simulink model "DWPT_DD_4section_100V"  (R2026b)
settings: Solver=ode3  StopTime=.050  FixedStep=Ts
model workspace (MAT data in the model file):
  Cf = 1e-07
  Cout = 0.0022
  Cp = 2.26347657939e-08
  Cs = 1.84570546919e-08
  ESRf = 0.003
  ESRp = 0.005
  ESRs = 0.005
  Goff = 1e-08
  Ki = 15
  Kp = 0.012
  Lf = 4.05284734569e-06
  Lmat = [2.19582561429e-05  -4.36667057516e-08  -2.64487562385e-10  -2.91825501354e-11  1.6585415982e-06; -4.36667057516e-08  2.19582561429e-05  -4.36667057516e-08  -2.64487562385e-10  1.6585415982e-06; -2.64487562385e-10  -4.36667057516e-08  2.19582561429e-05  -4.36667057516e-08  -1.36008982282e-09; -2.91825501354e-11  -2.64487562385e-10  -4.36667057516e-08  2.19582561429e-05  -7.55518058561e-11; 1.6585415982e-06  1.6585415982e-06  -1.36008982282e-09  -7.55518058561e-11  2.19582561429e-05]
  QossTx = 1.45e-07
  RL = 3
  Rcoil = 0.019579897138
  Rf = 0.006
  RonSR = 0.0032
  RonTx = 0.008
  Ts = 1e-08
  Vdc = 100
  Vtarget = 60
  bodyRon = 0.01
  bodyRonTx = 0.008
  bodyVf = 0.8
  bodyVfTx = 2
  deadTime = 2e-08
  f = 250000
  initialOutputVoltage = 0
  position = 0.9144
  softStart = 0.02
  srDeadTime = 4e-08
  srEnabled = 1
  srThreshold = 0.25
  transitionTime = 5e-09
  u_nom = [0.744962860955 0.744962860955 0 0]
libraries: fl_lib x52, nesl_utility x42, ee_lib x20, ddtrack_lib x1
(part 1 of 4)
settings Model: Creator=rithvik  LastModifiedBy=rithvik
settings DataIOCC: SignalLogging=off
settings SimscapeCC: SimscapeLogType=all  SimscapeNominalValues="[{\"value\":\"1\",\"unit\":\"A\"},{\"value\":\"1\",\"unit\":\"bar\"},{\"value\":\"1\",\"unit\":\"cm^2\"},{\"value\":\"1\",\"unit\":\"cm^3/s\"},{\"value\":\"1\",\"unit\":\"kJ/kg\"},{\"value\":\"1\",\"unit\":\"kW\"},{\"value\":\"1\",\"unit\":\"l\"},{\"value\":\"1\",\"unit\":\"N\"},{\"value\":\"1\",\"unit\":\"N*m\"},{\"value\":\"1\",\"unit\":\"V\"},{\"value\":\"0.001\",\"unit\":\"Wb\"}]"  SimscapeUseEnergyAccounting=off

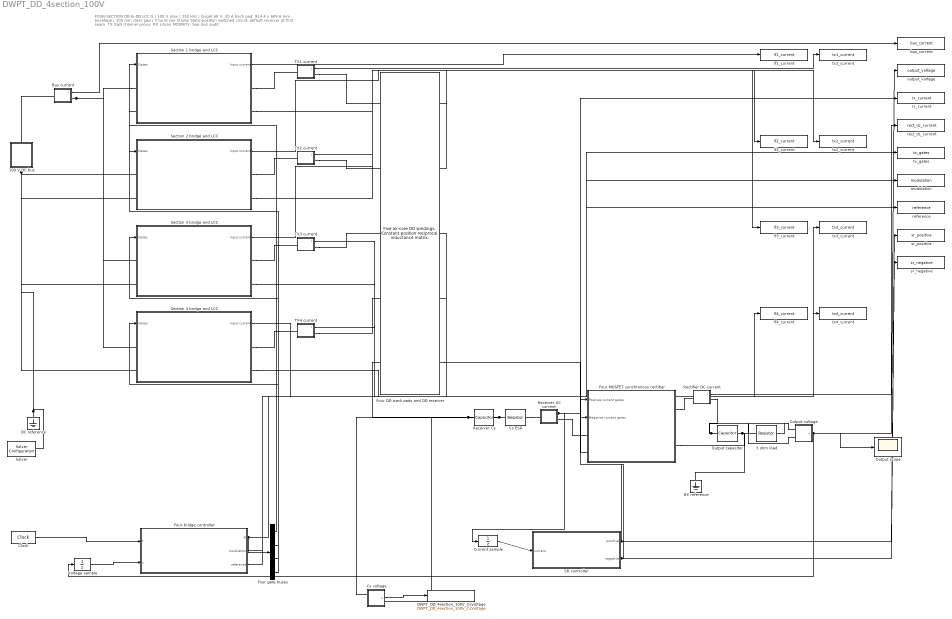
== system DWPT_DD_4section_100V ==
  note: FOUR-SECTION DD-to-DD LCC-S | 100 V max | 250 kHz | target 60 V, 20 A
      | Each pad: 914.4 x 609.6 mm envelope | 100 mm clear gap | 3 turns per D lobe
      | Static-position switched circuit; default receiver at first seam. TX GaN channel proxy; RX silicon MOSFETs. See loss audit.
  100 V DC bus : Subsystem
      settings: OpenFcn=elec.conv.unmask(gcb);
  3 ohm load : fl_lib/Electrical/Electrical Elements/Resistor  R=RL Ohm  i_specify=off  i_priority=None  i=0 A  i_nominal_specify=off  i_nominal_value=1  i_nominal_unit=A  v_specify=off  v_priority=None  v=0 V  v_nominal_specify=off  v_nominal_value=1  v_nominal_unit=V
  Bus current : Subsystem
      settings: OpenFcn=elec.conv.unmask(gcb);
  Clock : DigitalClock  SampleTime=Ts
  Cs ESR : fl_lib/Electrical/Electrical Elements/Resistor  R=ESRs Ohm  i_specify=off  i_priority=None  i=0 A  i_nominal_specify=off  i_nominal_value=1  i_nominal_unit=A  v_specify=off  v_priority=None  v=0 V  v_nominal_specify=off  v_nominal_value=1  v_nominal_unit=V
  Cs voltage : Subsystem
      settings: OpenFcn=elec.conv.unmask(gcb);
  Current sample : UnitDelay  SampleTime=Ts
  DC reference : fl_lib/Electrical/Electrical Elements/Electrical Reference
  DWPT_DD_4section_100V_CsVoltage : ToWorkspace  VariableName=DWPT_DD_4section_100V_CsVoltage  SaveFormat=Timeseries  SampleTime=-1
      settings: Decimation=max(1,round(20e-9/Ts))
  Four DD track pads and DD receiver : ddtrack_lib/Five air-core DD windings. Constant-position reciprocal inductance matrix.  Lmat=Lmat H  Rw=Rcoil Ohm  i1_specify=off  i1_priority=High  i1=0 A  i1_nominal_specify=off  i1_nominal_value=1  i1_nominal_unit=A  i2_specify=off  i2_priority=High  i2=0 A  i2_nominal_specify=off  i2_nominal_value=1  i2_nominal_unit=A  i3_specify=off  i3_priority=High  i3=0 A  i3_nominal_specify=off  i3_nominal_value=1  i3_nominal_unit=A  i4_specify=off  i4_priority=High  i4=0 A  i4_nominal_specify=off  i4_nominal_value=1  i4_nominal_unit=A  i5_specify=off  i5_priority=High  i5=0 A  i5_nominal_specify=off  i5_nominal_value=1  i5_nominal_unit=A
  Four MOSFET synchronous rectifier : Subsystem
  Four bridge controller : MATLAB Function  TreatAsAtomicUnit=on
  Four gate buses : Demux  Outputs=[4 4 4 4]
  Output capacitor : fl_lib/Electrical/Electrical Elements/Capacitor  c=Cout F  r=1e-6 Ohm  g=0 1/Ohm  i_specify=off  i_priority=None  i=0 A  i_nominal_specify=off  i_nominal_value=1  i_nominal_unit=A  v_specify=off  v_priority=None  v=0 V  v_nominal_specify=off  v_nominal_value=1  v_nominal_unit=V  vc_specify=on  vc_priority=High  vc=initialOutputVoltage V  vc_nominal_specify=off  vc_nominal_value=1  vc_nominal_unit=V
  Output scope : Scope
  Output voltage : Subsystem
      settings: OpenFcn=elec.conv.unmask(gcb);
  RX reference : fl_lib/Electrical/Electrical Elements/Electrical Reference
  Receiver AC current : Subsystem
      settings: OpenFcn=elec.conv.unmask(gcb);
  Receiver Cs : fl_lib/Electrical/Electrical Elements/Capacitor  c=Cs F  r=1e-6 Ohm  g=0 1/Ohm  i_specify=off  i_priority=None  i=0 A  i_nominal_specify=off  i_nominal_value=1  i_nominal_unit=A  v_specify=off  v_priority=None  v=0 V  v_nominal_specify=off  v_nominal_value=1  v_nominal_unit=V  vc_specify=on  vc_priority=High  vc=0 V  vc_nominal_specify=off  vc_nominal_value=1  vc_nominal_unit=V
  Rectifier DC current : Subsystem
      settings: OpenFcn=elec.conv.unmask(gcb);
  SR controller : MATLAB Function  TreatAsAtomicUnit=on
  Section 1 bridge and LCC : Subsystem
  Section 2 bridge and LCC : Subsystem
  Section 3 bridge and LCC : Subsystem
  Section 4 bridge and LCC : Subsystem
  Solver : nesl_utility/Solver Configuration  PhysicalDomain=network_engine_domain  SubClassName=solver  LeftPortType=input  RightPortType=generic  Tones=[]  Harmonics=[]  SimulateNoise=off  Profile=off  UseLocalSampling=off  EnableSwitchedLinearOptims=on  FrequencyDomain=off  UseCCode=off  RelTol=0.001  AbsTol=0.001  MinStep=1e-09  ToWorkspace=off  RevertToSquareIcSolve=off  NumHomotopyIterations=100  PhasorMode=off  PhasorModeNumHarmonics=1  ConsistencySolver=NEWTON_XTOL_AFTER_FTOL  CanonicalOrdering=CANONICAL  OptimizeIntermediates=OPTIMIZED  MulticoreSolverChoice=BACKWARD_EULER  IndexReductionMethod=DerivativeReplacement  DoDC=off  ResidualTolerance=1e-09  ConsistencyTolSource=GLOBAL  ConsistencyAbsTol=0.001  ConsistencyRelTol=0.001  ConsistencyTolFactor=0.001  UseLocalSolver=on  LocalSolverChoice=NE_TRAPEZOIDAL_ADVANCER  ResolveIndetEquations=on  FunctionEvalNumThread=1  LocalSolverSampleTime=Ts  DoFixedCost=off  MaxNonlinIter=3  MaxModeIter=2  ComputeImpulses=off  ImpulseIterations=2  LinearAlgebra=auto  LinearAlgebraNumThread=0  EquationFormulation=NE_TIME_EF  DelaysMemoryBudget=1024  AutomaticFiltering=on  FilteringTimeConstant=0.001  PartitionStorageMethod=AS_NEEDED  PartitionMemoryBudget=1024  PartitionMethod=BALANCED  MultibodyUseLocalSolver=off  MultibodyLocalSolverChoice=ODE1  MultibodyLocalSolverSampleTime=0.001
  TX1 current : Subsystem
      settings: OpenFcn=elec.conv.unmask(gcb);
  TX2 current : Subsystem
      settings: OpenFcn=elec.conv.unmask(gcb);
  TX3 current : Subsystem
      settings: OpenFcn=elec.conv.unmask(gcb);
  TX4 current : Subsystem
      settings: OpenFcn=elec.conv.unmask(gcb);
  Voltage sample : UnitDelay  SampleTime=Ts
  bus_current : ToWorkspace  VariableName=bus_current  SaveFormat=Timeseries  SampleTime=-1
  lf1_current : ToWorkspace  VariableName=lf1_current  SaveFormat=Timeseries  SampleTime=-1
      settings: Decimation=max(1,round(20e-9/Ts))
  lf2_current : ToWorkspace  VariableName=lf2_current  SaveFormat=Timeseries  SampleTime=-1
      settings: Decimation=max(1,round(20e-9/Ts))
  lf3_current : ToWorkspace  VariableName=lf3_current  SaveFormat=Timeseries  SampleTime=-1
      settings: Decimation=max(1,round(20e-9/Ts))
  lf4_current : ToWorkspace  VariableName=lf4_current  SaveFormat=Timeseries  SampleTime=-1
      settings: Decimation=max(1,round(20e-9/Ts))
  modulation : ToWorkspace  VariableName=modulation  SaveFormat=Timeseries  SampleTime=-1
      settings: Decimation=max(1,round(20e-9/Ts))
  output_voltage : ToWorkspace  VariableName=output_voltage  SaveFormat=Timeseries  SampleTime=-1
      settings: Decimation=max(1,round(20e-9/Ts))
  rect_dc_current : ToWorkspace  VariableName=rect_dc_current  SaveFormat=Timeseries  SampleTime=-1
      settings: Decimation=max(1,round(20e-9/Ts))
  reference : ToWorkspace  VariableName=reference  SaveFormat=Timeseries  SampleTime=-1
      settings: Decimation=max(1,round(20e-9/Ts))
  rx_current : ToWorkspace  VariableName=rx_current  SaveFormat=Timeseries  SampleTime=-1
      settings: Decimation=max(1,round(20e-9/Ts))
  sr_negative : ToWorkspace  VariableName=sr_negative  SaveFormat=Timeseries  SampleTime=-1
      settings: Decimation=max(1,round(20e-9/Ts))
  sr_positive : ToWorkspace  VariableName=sr_positive  SaveFormat=Timeseries  SampleTime=-1
      settings: Decimation=max(1,round(20e-9/Ts))
  tx1_current : ToWorkspace  VariableName=tx1_current  SaveFormat=Timeseries  SampleTime=-1
      settings: Decimation=max(1,round(20e-9/Ts))
  tx2_current : ToWorkspace  VariableName=tx2_current  SaveFormat=Timeseries  SampleTime=-1
      settings: Decimation=max(1,round(20e-9/Ts))
  tx3_current : ToWorkspace  VariableName=tx3_current  SaveFormat=Timeseries  SampleTime=-1
      settings: Decimation=max(1,round(20e-9/Ts))
  tx4_current : ToWorkspace  VariableName=tx4_current  SaveFormat=Timeseries  SampleTime=-1
      settings: Decimation=max(1,round(20e-9/Ts))
  tx_gates : ToWorkspace  VariableName=tx_gates  SaveFormat=Timeseries  SampleTime=-1
      settings: Decimation=max(1,round(20e-9/Ts))
  wires:
  Section 1 bridge and LCC/1(Input current) -> lf1_current/1
  TX1 current/1(i) -> tx1_current/1
  Section 2 bridge and LCC/1(Input current) -> lf2_current/1
  TX2 current/1(i) -> tx2_current/1
  Section 3 bridge and LCC/1(Input current) -> lf3_current/1
  TX3 current/1(i) -> tx3_current/1
  Section 4 bridge and LCC/1(Input current) -> lf4_current/1
  TX4 current/1(i) -> tx4_current/1
  Clock/1 -> Four bridge controller/1(t)
  Output voltage/1(v) -> Voltage sample/1, output_voltage/1, Output scope/1
  Voltage sample/1 -> Four bridge controller/2(v)
  Four bridge controller/1(g) -> Four gate buses/1, tx_gates/1
  Four gate buses/1 -> Section 1 bridge and LCC/1(Gates)
  Four gate buses/2 -> Section 2 bridge and LCC/1(Gates)
  Four gate buses/3 -> Section 3 bridge and LCC/1(Gates)
  Four gate buses/4 -> Section 4 bridge and LCC/1(Gates)
  Receiver AC current/1(i) -> Current sample/1, rx_current/1
  Current sample/1 -> SR controller/1(current)
  SR controller/1(positive) -> Four MOSFET synchronous rectifier/1(Positive current gates), sr_positive/1
  SR controller/2(negative) -> Four MOSFET synchronous rectifier/2(Negative current gates), sr_negative/1
  Bus current/1(i) -> bus_current/1
  Rectifier DC current/1(i) -> rect_dc_current/1
  Four bridge controller/2(modulation) -> modulation/1
  Four bridge controller/3(reference) -> reference/1
  Cs voltage/1(v) -> DWPT_DD_4section_100V_CsVoltage/1
  connections:
  100 V DC bus/RConn1 -- Bus current/LConn1
  DC reference/LConn1 -- 100 V DC bus/LConn1 -- Section 1 bridge and LCC/LConn2 -- Section 2 bridge and LCC/LConn2 -- Section 3 bridge and LCC/LConn2 -- Section 4 bridge and LCC/LConn2 -- Solver/RConn1
  Section 1 bridge and LCC/LConn1 -- Bus current/RConn1 -- Section 2 bridge and LCC/LConn1 -- Section 3 bridge and LCC/LConn1 -- Section 4 bridge and LCC/LConn1
  Section 1 bridge and LCC/RConn1 -- TX1 current/LConn1
  TX1 current/RConn1 -- Four DD track pads and DD receiver/LConn1
  Section 1 bridge and LCC/RConn2 -- Four DD track pads and DD receiver/RConn1
  Section 2 bridge and LCC/RConn1 -- TX2 current/LConn1
  TX2 current/RConn1 -- Four DD track pads and DD receiver/LConn2
  Section 2 bridge and LCC/RConn2 -- Four DD track pads and DD receiver/RConn2
  Section 3 bridge and LCC/RConn1 -- TX3 current/LConn1
  TX3 current/RConn1 -- Four DD track pads and DD receiver/LConn3
  Section 3 bridge and LCC/RConn2 -- Four DD track pads and DD receiver/RConn3
  Section 4 bridge and LCC/RConn1 -- TX4 current/LConn1
  TX4 current/RConn1 -- Four DD track pads and DD receiver/LConn4
  Section 4 bridge and LCC/RConn2 -- Four DD track pads and DD receiver/RConn4
  Receiver Cs/LConn1 -- Four DD track pads and DD receiver/LConn5 -- Cs voltage/LConn1
  Cs ESR/LConn1 -- Receiver Cs/RConn1 -- Cs voltage/LConn2
  Cs ESR/RConn1 -- Receiver AC current/LConn1
  Receiver AC current/RConn1 -- Four MOSFET synchronous rectifier/LConn1
  Four DD track pads and DD receiver/RConn5 -- Four MOSFET synchronous rectifier/LConn2
  Four MOSFET synchronous rectifier/RConn1 -- Rectifier DC current/LConn1
  Rectifier DC current/RConn1 -- 3 ohm load/LConn1 -- Output capacitor/LConn1 -- Output voltage/LConn1
  Four MOSFET synchronous rectifier/RConn2 -- 3 ohm load/RConn1 -- RX reference/LConn1 -- Output capacitor/RConn1 -- Output voltage/LConn2

== system DWPT_DD_4section_100V/100 V DC bus ==
  DC Voltage Source : fl_lib/Electrical/Electrical Sources/DC Voltage Source  v0=Vdc V
  - : PMIOPort  Side=Left
  + : PMIOPort  Port=2  Side=Right
  connections:
  DC Voltage Source/LConn1 -- +/RConn1
  DC Voltage Source/RConn1 -- -/RConn1

== system DWPT_DD_4section_100V/Bus current ==
  Current Sensor : fl_lib/Electrical/Electrical Sensors/Current Sensor
  PS-Simulink Converter : nesl_utility/PS-Simulink Converter  PhysicalDomain=network_engine_domain  SubClassName=ps_output  LeftPortType=input  RightPortType=output  PseudoPeriodic=off  Frequencies=[]  VectorFormat=1-D array  Unit=A  AffineConversion=off
  + : PMIOPort  Side=Left
  - : PMIOPort  Port=2  Side=Right
  i : Outport  VectorParamsAs1DForOutWhenUnconnected=off
  wires:
  PS-Simulink Converter/1 -> i/1
  connections:
  PS-Simulink Converter/LConn1 -- Current Sensor/RConn1
  -/RConn1 -- Current Sensor/RConn2
  +/RConn1 -- Current Sensor/LConn1

== system DWPT_DD_4section_100V/Cs voltage ==
  PS-Simulink Converter : nesl_utility/PS-Simulink Converter  PhysicalDomain=network_engine_domain  SubClassName=ps_output  LeftPortType=input  RightPortType=output  PseudoPeriodic=off  Frequencies=[]  VectorFormat=1-D array  Unit=V  AffineConversion=off
  Voltage Sensor : fl_lib/Electrical/Electrical Sensors/Voltage Sensor
  + : PMIOPort  Side=Left
  - : PMIOPort  Port=2  Side=Left
  v : Outport  VectorParamsAs1DForOutWhenUnconnected=off
  wires:
  PS-Simulink Converter/1 -> v/1
  connections:
  +/RConn1 -- Voltage Sensor/LConn1
  -/RConn1 -- Voltage Sensor/RConn2
  PS-Simulink Converter/LConn1 -- Voltage Sensor/RConn1

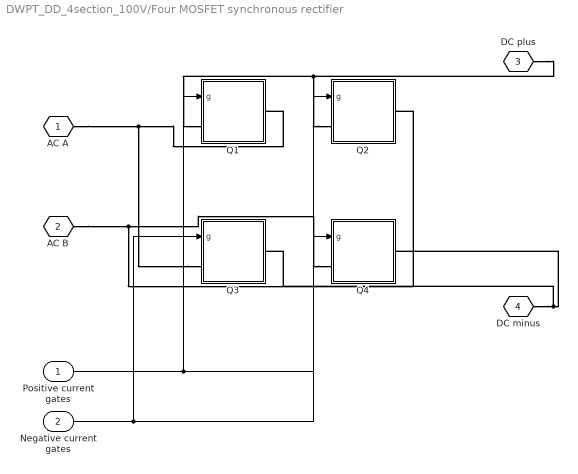
== system DWPT_DD_4section_100V/Four MOSFET synchronous rectifier ==
  Positive current gates : Inport
  Negative current gates : Inport  Port=2
  Q1 : Subsystem
  Q2 : Subsystem
  Q3 : Subsystem
  Q4 : Subsystem
  AC A : PMIOPort  Side=Left
  AC B : PMIOPort  Port=2  Side=Left
  DC plus : PMIOPort  Port=3  Side=Right
  DC minus : PMIOPort  Port=4  Side=Right
  wires:
  Negative current gates/1 -> Q3/1(g), Q2/1(g)
  Positive current gates/1 -> Q4/1(g), Q1/1(g)
  connections:
  Q4/RConn1 -- DC minus/RConn1 -- Q3/RConn1
  Q4/LConn1 -- AC B/RConn1 -- Q2/RConn1
  Q3/LConn1 -- AC A/RConn1 -- Q1/RConn1
  Q2/LConn1 -- DC plus/RConn1 -- Q1/LConn1

== system DWPT_DD_4section_100V/Output voltage ==
  PS-Simulink Converter : nesl_utility/PS-Simulink Converter  PhysicalDomain=network_engine_domain  SubClassName=ps_output  LeftPortType=input  RightPortType=output  PseudoPeriodic=off  Frequencies=[]  VectorFormat=1-D array  Unit=V  AffineConversion=off
  Voltage Sensor : fl_lib/Electrical/Electrical Sensors/Voltage Sensor
  + : PMIOPort  Side=Left
  - : PMIOPort  Port=2  Side=Left
  v : Outport  VectorParamsAs1DForOutWhenUnconnected=off
  wires:
  PS-Simulink Converter/1 -> v/1
  connections:
  +/RConn1 -- Voltage Sensor/LConn1
  -/RConn1 -- Voltage Sensor/RConn2
  PS-Simulink Converter/LConn1 -- Voltage Sensor/RConn1

== system DWPT_DD_4section_100V/Receiver AC current ==
  Current Sensor : fl_lib/Electrical/Electrical Sensors/Current Sensor
  PS-Simulink Converter : nesl_utility/PS-Simulink Converter  PhysicalDomain=network_engine_domain  SubClassName=ps_output  LeftPortType=input  RightPortType=output  PseudoPeriodic=off  Frequencies=[]  VectorFormat=1-D array  Unit=A  AffineConversion=off
  + : PMIOPort  Side=Left
  - : PMIOPort  Port=2  Side=Right
  i : Outport  VectorParamsAs1DForOutWhenUnconnected=off
  wires:
  PS-Simulink Converter/1 -> i/1
  connections:
  PS-Simulink Converter/LConn1 -- Current Sensor/RConn1
  -/RConn1 -- Current Sensor/RConn2
  +/RConn1 -- Current Sensor/LConn1

== system DWPT_DD_4section_100V/Rectifier DC current ==
  Current Sensor : fl_lib/Electrical/Electrical Sensors/Current Sensor
  PS-Simulink Converter : nesl_utility/PS-Simulink Converter  PhysicalDomain=network_engine_domain  SubClassName=ps_output  LeftPortType=input  RightPortType=output  PseudoPeriodic=off  Frequencies=[]  VectorFormat=1-D array  Unit=A  AffineConversion=off
  + : PMIOPort  Side=Left
  - : PMIOPort  Port=2  Side=Right
  i : Outport  VectorParamsAs1DForOutWhenUnconnected=off
  wires:
  PS-Simulink Converter/1 -> i/1
  connections:
  PS-Simulink Converter/LConn1 -- Current Sensor/RConn1
  -/RConn1 -- Current Sensor/RConn2
  +/RConn1 -- Current Sensor/LConn1

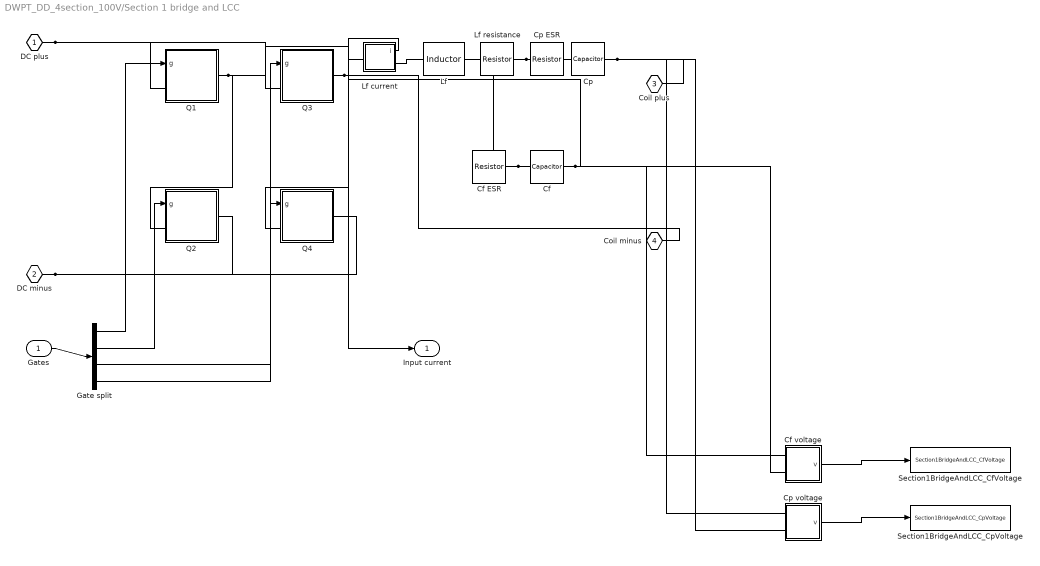
== system DWPT_DD_4section_100V/Section 1 bridge and LCC ==
  Gates : Inport
  Cf : fl_lib/Electrical/Electrical Elements/Capacitor  c=Cf F  r=1e-6 Ohm  g=0 1/Ohm  i_specify=off  i_priority=None  i=0 A  i_nominal_specify=off  i_nominal_value=1  i_nominal_unit=A  v_specify=off  v_priority=None  v=0 V  v_nominal_specify=off  v_nominal_value=1  v_nominal_unit=V  vc_specify=on  vc_priority=High  vc=0 V  vc_nominal_specify=off  vc_nominal_value=1  vc_nominal_unit=V
  Cf ESR : fl_lib/Electrical/Electrical Elements/Resistor  R=ESRf Ohm  i_specify=off  i_priority=None  i=0 A  i_nominal_specify=off  i_nominal_value=1  i_nominal_unit=A  v_specify=off  v_priority=None  v=0 V  v_nominal_specify=off  v_nominal_value=1  v_nominal_unit=V
  Cf voltage : Subsystem
      settings: OpenFcn=elec.conv.unmask(gcb);
  Cp : fl_lib/Electrical/Electrical Elements/Capacitor  c=Cp F  r=1e-6 Ohm  g=0 1/Ohm  i_specify=off  i_priority=None  i=0 A  i_nominal_specify=off  i_nominal_value=1  i_nominal_unit=A  v_specify=off  v_priority=None  v=0 V  v_nominal_specify=off  v_nominal_value=1  v_nominal_unit=V  vc_specify=on  vc_priority=High  vc=0 V  vc_nominal_specify=off  vc_nominal_value=1  vc_nominal_unit=V
  Cp ESR : fl_lib/Electrical/Electrical Elements/Resistor  R=ESRp Ohm  i_specify=off  i_priority=None  i=0 A  i_nominal_specify=off  i_nominal_value=1  i_nominal_unit=A  v_specify=off  v_priority=None  v=0 V  v_nominal_specify=off  v_nominal_value=1  v_nominal_unit=V
  Cp voltage : Subsystem
      settings: OpenFcn=elec.conv.unmask(gcb);
  Gate split : Demux
  Lf : fl_lib/Electrical/Electrical Elements/Inductor  l=Lf H  r=0 Ohm  g=1e-9 1/Ohm  i_specify=off  i_priority=None  i=0 A  i_nominal_specify=off  i_nominal_value=1  i_nominal_unit=A  v_specify=off  v_priority=None  v=0 V  v_nominal_specify=off  v_nominal_value=1  v_nominal_unit=V  i_L_specify=on  i_L_priority=High  i_L=0 A  i_L_nominal_specify=off  i_L_nominal_value=1  i_L_nominal_unit=A
  Lf current : Subsystem
      settings: OpenFcn=elec.conv.unmask(gcb);
  Lf resistance : fl_lib/Electrical/Electrical Elements/Resistor  R=Rf Ohm  i_specify=off  i_priority=None  i=0 A  i_nominal_specify=off  i_nominal_value=1  i_nominal_unit=A  v_specify=off  v_priority=None  v=0 V  v_nominal_specify=off  v_nominal_value=1  v_nominal_unit=V
  Q1 : Subsystem
  Q2 : Subsystem
  Q3 : Subsystem
  Q4 : Subsystem
  Section1BridgeAndLCC_CfVoltage : ToWorkspace  VariableName=Section1BridgeAndLCC_CfVoltage  SaveFormat=Timeseries  SampleTime=-1
      settings: Decimation=max(1,round(20e-9/Ts))
  Section1BridgeAndLCC_CpVoltage : ToWorkspace  VariableName=Section1BridgeAndLCC_CpVoltage  SaveFormat=Timeseries  SampleTime=-1
      settings: Decimation=max(1,round(20e-9/Ts))
  DC plus : PMIOPort  Side=Left
  DC minus : PMIOPort  Port=2  Side=Left
  Coil plus : PMIOPort  Port=3  Side=Right
  Coil minus : PMIOPort  Port=4  Side=Right
  Input current : Outport
  wires:
  Gates/1 -> Gate split/1
  Gate split/1 -> Q1/1(g)
  Gate split/2 -> Q2/1(g)
  Gate split/3 -> Q3/1(g)
  Gate split/4 -> Q4/1(g)
  Lf current/1(i) -> Input current/1
  Cf voltage/1(v) -> Section1BridgeAndLCC_CfVoltage/1
  Cp voltage/1(v) -> Section1BridgeAndLCC_CpVoltage/1
  connections:
  Q1/LConn1 -- DC plus/RConn1 -- Q3/LConn1
  Q2/RConn1 -- DC minus/RConn1 -- Q4/RConn1
  Q2/LConn1 -- Q1/RConn1 -- Lf current/LConn1
  Q4/LConn1 -- Q3/RConn1 -- Cf/RConn1 -- Cf voltage/LConn2 -- Coil minus/RConn1
  Lf current/RConn1 -- Lf/LConn1
  Lf/RConn1 -- Lf resistance/LConn1
  Cp ESR/LConn1 -- Lf resistance/RConn1 -- Cf ESR/LConn1
  Cp/LConn1 -- Cp ESR/RConn1 -- Cp voltage/LConn1
  Coil plus/RConn1 -- Cp/RConn1 -- Cp voltage/LConn2
  Cf/LConn1 -- Cf ESR/RConn1 -- Cf voltage/LConn1

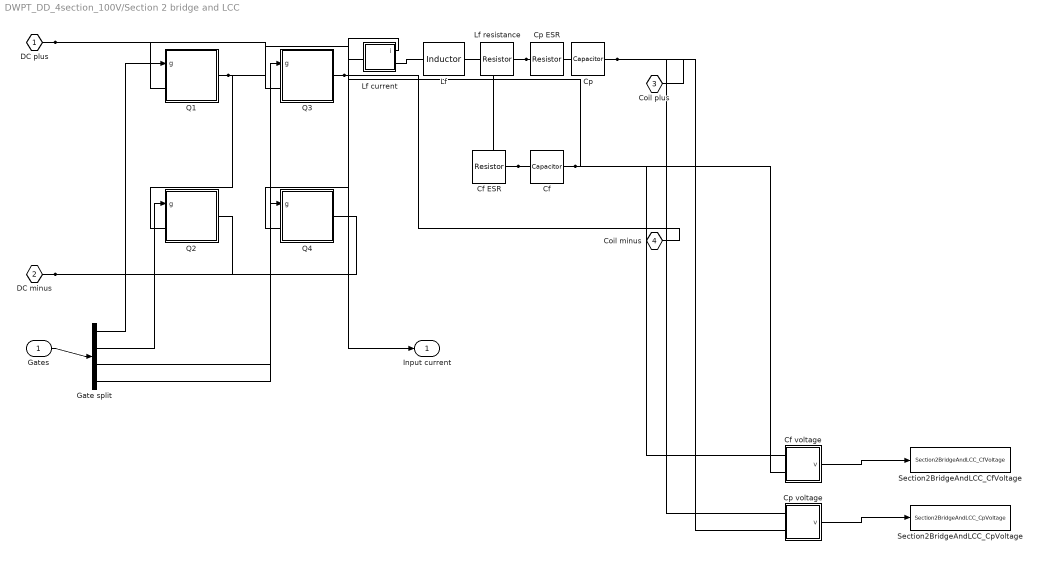
== system DWPT_DD_4section_100V/Section 2 bridge and LCC ==
  Gates : Inport
  Cf : fl_lib/Electrical/Electrical Elements/Capacitor  c=Cf F  r=1e-6 Ohm  g=0 1/Ohm  i_specify=off  i_priority=None  i=0 A  i_nominal_specify=off  i_nominal_value=1  i_nominal_unit=A  v_specify=off  v_priority=None  v=0 V  v_nominal_specify=off  v_nominal_value=1  v_nominal_unit=V  vc_specify=on  vc_priority=High  vc=0 V  vc_nominal_specify=off  vc_nominal_value=1  vc_nominal_unit=V
  Cf ESR : fl_lib/Electrical/Electrical Elements/Resistor  R=ESRf Ohm  i_specify=off  i_priority=None  i=0 A  i_nominal_specify=off  i_nominal_value=1  i_nominal_unit=A  v_specify=off  v_priority=None  v=0 V  v_nominal_specify=off  v_nominal_value=1  v_nominal_unit=V
  Cf voltage : Subsystem
      settings: OpenFcn=elec.conv.unmask(gcb);
  Cp : fl_lib/Electrical/Electrical Elements/Capacitor  c=Cp F  r=1e-6 Ohm  g=0 1/Ohm  i_specify=off  i_priority=None  i=0 A  i_nominal_specify=off  i_nominal_value=1  i_nominal_unit=A  v_specify=off  v_priority=None  v=0 V  v_nominal_specify=off  v_nominal_value=1  v_nominal_unit=V  vc_specify=on  vc_priority=High  vc=0 V  vc_nominal_specify=off  vc_nominal_value=1  vc_nominal_unit=V
  Cp ESR : fl_lib/Electrical/Electrical Elements/Resistor  R=ESRp Ohm  i_specify=off  i_priority=None  i=0 A  i_nominal_specify=off  i_nominal_value=1  i_nominal_unit=A  v_specify=off  v_priority=None  v=0 V  v_nominal_specify=off  v_nominal_value=1  v_nominal_unit=V
  Cp voltage : Subsystem
      settings: OpenFcn=elec.conv.unmask(gcb);
  Gate split : Demux
  Lf : fl_lib/Electrical/Electrical Elements/Inductor  l=Lf H  r=0 Ohm  g=1e-9 1/Ohm  i_specify=off  i_priority=None  i=0 A  i_nominal_specify=off  i_nominal_value=1  i_nominal_unit=A  v_specify=off  v_priority=None  v=0 V  v_nominal_specify=off  v_nominal_value=1  v_nominal_unit=V  i_L_specify=on  i_L_priority=High  i_L=0 A  i_L_nominal_specify=off  i_L_nominal_value=1  i_L_nominal_unit=A
  Lf current : Subsystem
      settings: OpenFcn=elec.conv.unmask(gcb);
  Lf resistance : fl_lib/Electrical/Electrical Elements/Resistor  R=Rf Ohm  i_specify=off  i_priority=None  i=0 A  i_nominal_specify=off  i_nominal_value=1  i_nominal_unit=A  v_specify=off  v_priority=None  v=0 V  v_nominal_specify=off  v_nominal_value=1  v_nominal_unit=V
  Q1 : Subsystem
  Q2 : Subsystem
  Q3 : Subsystem
  Q4 : Subsystem
  Section2BridgeAndLCC_CfVoltage : ToWorkspace  VariableName=Section2BridgeAndLCC_CfVoltage  SaveFormat=Timeseries  SampleTime=-1
      settings: Decimation=max(1,round(20e-9/Ts))
  Section2BridgeAndLCC_CpVoltage : ToWorkspace  VariableName=Section2BridgeAndLCC_CpVoltage  SaveFormat=Timeseries  SampleTime=-1
      settings: Decimation=max(1,round(20e-9/Ts))
  DC plus : PMIOPort  Side=Left
  DC minus : PMIOPort  Port=2  Side=Left
  Coil plus : PMIOPort  Port=3  Side=Right
  Coil minus : PMIOPort  Port=4  Side=Right
  Input current : Outport
  wires:
  Gates/1 -> Gate split/1
  Gate split/1 -> Q1/1(g)
  Gate split/2 -> Q2/1(g)
  Gate split/3 -> Q3/1(g)
  Gate split/4 -> Q4/1(g)
  Lf current/1(i) -> Input current/1
  Cf voltage/1(v) -> Section2BridgeAndLCC_CfVoltage/1
  Cp voltage/1(v) -> Section2BridgeAndLCC_CpVoltage/1
  connections:
  Q1/LConn1 -- DC plus/RConn1 -- Q3/LConn1
  Q2/RConn1 -- DC minus/RConn1 -- Q4/RConn1
  Q2/LConn1 -- Q1/RConn1 -- Lf current/LConn1
  Q4/LConn1 -- Q3/RConn1 -- Cf/RConn1 -- Cf voltage/LConn2 -- Coil minus/RConn1
  Lf current/RConn1 -- Lf/LConn1
  Lf/RConn1 -- Lf resistance/LConn1
  Cp ESR/LConn1 -- Lf resistance/RConn1 -- Cf ESR/LConn1
  Cp/LConn1 -- Cp ESR/RConn1 -- Cp voltage/LConn1
  Coil plus/RConn1 -- Cp/RConn1 -- Cp voltage/LConn2
  Cf/LConn1 -- Cf ESR/RConn1 -- Cf voltage/LConn1

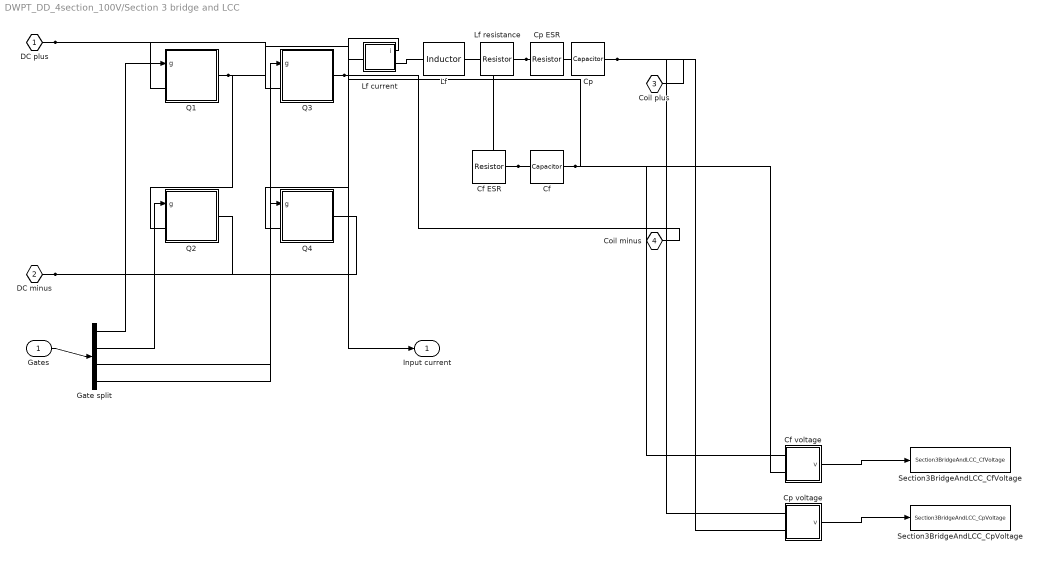
== system DWPT_DD_4section_100V/Section 3 bridge and LCC ==
  Gates : Inport
  Cf : fl_lib/Electrical/Electrical Elements/Capacitor  c=Cf F  r=1e-6 Ohm  g=0 1/Ohm  i_specify=off  i_priority=None  i=0 A  i_nominal_specify=off  i_nominal_value=1  i_nominal_unit=A  v_specify=off  v_priority=None  v=0 V  v_nominal_specify=off  v_nominal_value=1  v_nominal_unit=V  vc_specify=on  vc_priority=High  vc=0 V  vc_nominal_specify=off  vc_nominal_value=1  vc_nominal_unit=V
  Cf ESR : fl_lib/Electrical/Electrical Elements/Resistor  R=ESRf Ohm  i_specify=off  i_priority=None  i=0 A  i_nominal_specify=off  i_nominal_value=1  i_nominal_unit=A  v_specify=off  v_priority=None  v=0 V  v_nominal_specify=off  v_nominal_value=1  v_nominal_unit=V
  Cf voltage : Subsystem
      settings: OpenFcn=elec.conv.unmask(gcb);
  Cp : fl_lib/Electrical/Electrical Elements/Capacitor  c=Cp F  r=1e-6 Ohm  g=0 1/Ohm  i_specify=off  i_priority=None  i=0 A  i_nominal_specify=off  i_nominal_value=1  i_nominal_unit=A  v_specify=off  v_priority=None  v=0 V  v_nominal_specify=off  v_nominal_value=1  v_nominal_unit=V  vc_specify=on  vc_priority=High  vc=0 V  vc_nominal_specify=off  vc_nominal_value=1  vc_nominal_unit=V
  Cp ESR : fl_lib/Electrical/Electrical Elements/Resistor  R=ESRp Ohm  i_specify=off  i_priority=None  i=0 A  i_nominal_specify=off  i_nominal_value=1  i_nominal_unit=A  v_specify=off  v_priority=None  v=0 V  v_nominal_specify=off  v_nominal_value=1  v_nominal_unit=V
  Cp voltage : Subsystem
      settings: OpenFcn=elec.conv.unmask(gcb);
  Gate split : Demux
  Lf : fl_lib/Electrical/Electrical Elements/Inductor  l=Lf H  r=0 Ohm  g=1e-9 1/Ohm  i_specify=off  i_priority=None  i=0 A  i_nominal_specify=off  i_nominal_value=1  i_nominal_unit=A  v_specify=off  v_priority=None  v=0 V  v_nominal_specify=off  v_nominal_value=1  v_nominal_unit=V  i_L_specify=on  i_L_priority=High  i_L=0 A  i_L_nominal_specify=off  i_L_nominal_value=1  i_L_nominal_unit=A
  Lf current : Subsystem
      settings: OpenFcn=elec.conv.unmask(gcb);
  Lf resistance : fl_lib/Electrical/Electrical Elements/Resistor  R=Rf Ohm  i_specify=off  i_priority=None  i=0 A  i_nominal_specify=off  i_nominal_value=1  i_nominal_unit=A  v_specify=off  v_priority=None  v=0 V  v_nominal_specify=off  v_nominal_value=1  v_nominal_unit=V
  Q1 : Subsystem
  Q2 : Subsystem
  Q3 : Subsystem
  Q4 : Subsystem
  Section3BridgeAndLCC_CfVoltage : ToWorkspace  VariableName=Section3BridgeAndLCC_CfVoltage  SaveFormat=Timeseries  SampleTime=-1
      settings: Decimation=max(1,round(20e-9/Ts))
  Section3BridgeAndLCC_CpVoltage : ToWorkspace  VariableName=Section3BridgeAndLCC_CpVoltage  SaveFormat=Timeseries  SampleTime=-1
      settings: Decimation=max(1,round(20e-9/Ts))
  DC plus : PMIOPort  Side=Left
  DC minus : PMIOPort  Port=2  Side=Left
  Coil plus : PMIOPort  Port=3  Side=Right
  Coil minus : PMIOPort  Port=4  Side=Right
  Input current : Outport
  wires:
  Gates/1 -> Gate split/1
  Gate split/1 -> Q1/1(g)
  Gate split/2 -> Q2/1(g)
  Gate split/3 -> Q3/1(g)
  Gate split/4 -> Q4/1(g)
  Lf current/1(i) -> Input current/1
  Cf voltage/1(v) -> Section3BridgeAndLCC_CfVoltage/1
  Cp voltage/1(v) -> Section3BridgeAndLCC_CpVoltage/1
  connections:
  Q1/LConn1 -- DC plus/RConn1 -- Q3/LConn1
  Q2/RConn1 -- DC minus/RConn1 -- Q4/RConn1
  Q2/LConn1 -- Q1/RConn1 -- Lf current/LConn1
  Q4/LConn1 -- Q3/RConn1 -- Cf/RConn1 -- Cf voltage/LConn2 -- Coil minus/RConn1
  Lf current/RConn1 -- Lf/LConn1
  Lf/RConn1 -- Lf resistance/LConn1
  Cp ESR/LConn1 -- Lf resistance/RConn1 -- Cf ESR/LConn1
  Cp/LConn1 -- Cp ESR/RConn1 -- Cp voltage/LConn1
  Coil plus/RConn1 -- Cp/RConn1 -- Cp voltage/LConn2
  Cf/LConn1 -- Cf ESR/RConn1 -- Cf voltage/LConn1

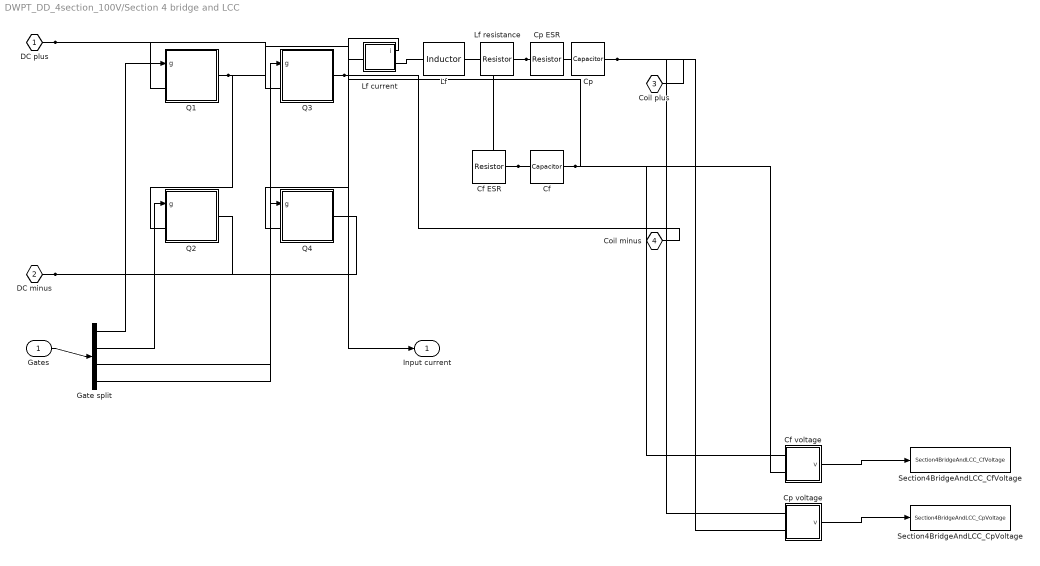
== system DWPT_DD_4section_100V/Section 4 bridge and LCC ==
  Gates : Inport
  Cf : fl_lib/Electrical/Electrical Elements/Capacitor  c=Cf F  r=1e-6 Ohm  g=0 1/Ohm  i_specify=off  i_priority=None  i=0 A  i_nominal_specify=off  i_nominal_value=1  i_nominal_unit=A  v_specify=off  v_priority=None  v=0 V  v_nominal_specify=off  v_nominal_value=1  v_nominal_unit=V  vc_specify=on  vc_priority=High  vc=0 V  vc_nominal_specify=off  vc_nominal_value=1  vc_nominal_unit=V
  Cf ESR : fl_lib/Electrical/Electrical Elements/Resistor  R=ESRf Ohm  i_specify=off  i_priority=None  i=0 A  i_nominal_specify=off  i_nominal_value=1  i_nominal_unit=A  v_specify=off  v_priority=None  v=0 V  v_nominal_specify=off  v_nominal_value=1  v_nominal_unit=V
  Cf voltage : Subsystem
      settings: OpenFcn=elec.conv.unmask(gcb);
  Cp : fl_lib/Electrical/Electrical Elements/Capacitor  c=Cp F  r=1e-6 Ohm  g=0 1/Ohm  i_specify=off  i_priority=None  i=0 A  i_nominal_specify=off  i_nominal_value=1  i_nominal_unit=A  v_specify=off  v_priority=None  v=0 V  v_nominal_specify=off  v_nominal_value=1  v_nominal_unit=V  vc_specify=on  vc_priority=High  vc=0 V  vc_nominal_specify=off  vc_nominal_value=1  vc_nominal_unit=V
  Cp ESR : fl_lib/Electrical/Electrical Elements/Resistor  R=ESRp Ohm  i_specify=off  i_priority=None  i=0 A  i_nominal_specify=off  i_nominal_value=1  i_nominal_unit=A  v_specify=off  v_priority=None  v=0 V  v_nominal_specify=off  v_nominal_value=1  v_nominal_unit=V
  Cp voltage : Subsystem
      settings: OpenFcn=elec.conv.unmask(gcb);
  Gate split : Demux
  Lf : fl_lib/Electrical/Electrical Elements/Inductor  l=Lf H  r=0 Ohm  g=1e-9 1/Ohm  i_specify=off  i_priority=None  i=0 A  i_nominal_specify=off  i_nominal_value=1  i_nominal_unit=A  v_specify=off  v_priority=None  v=0 V  v_nominal_specify=off  v_nominal_value=1  v_nominal_unit=V  i_L_specify=on  i_L_priority=High  i_L=0 A  i_L_nominal_specify=off  i_L_nominal_value=1  i_L_nominal_unit=A
  Lf current : Subsystem
      settings: OpenFcn=elec.conv.unmask(gcb);
  Lf resistance : fl_lib/Electrical/Electrical Elements/Resistor  R=Rf Ohm  i_specify=off  i_priority=None  i=0 A  i_nominal_specify=off  i_nominal_value=1  i_nominal_unit=A  v_specify=off  v_priority=None  v=0 V  v_nominal_specify=off  v_nominal_value=1  v_nominal_unit=V
  Q1 : Subsystem
  Q2 : Subsystem
  Q3 : Subsystem
  Q4 : Subsystem
  Section4BridgeAndLCC_CfVoltage : ToWorkspace  VariableName=Section4BridgeAndLCC_CfVoltage  SaveFormat=Timeseries  SampleTime=-1
      settings: Decimation=max(1,round(20e-9/Ts))
  Section4BridgeAndLCC_CpVoltage : ToWorkspace  VariableName=Section4BridgeAndLCC_CpVoltage  SaveFormat=Timeseries  SampleTime=-1
      settings: Decimation=max(1,round(20e-9/Ts))
  DC plus : PMIOPort  Side=Left
  DC minus : PMIOPort  Port=2  Side=Left
  Coil plus : PMIOPort  Port=3  Side=Right
  Coil minus : PMIOPort  Port=4  Side=Right
  Input current : Outport
  wires:
  Gates/1 -> Gate split/1
  Gate split/1 -> Q1/1(g)
  Gate split/2 -> Q2/1(g)
  Gate split/3 -> Q3/1(g)
  Gate split/4 -> Q4/1(g)
  Lf current/1(i) -> Input current/1
  Cf voltage/1(v) -> Section4BridgeAndLCC_CfVoltage/1
  Cp voltage/1(v) -> Section4BridgeAndLCC_CpVoltage/1
  connections:
  Q1/LConn1 -- DC plus/RConn1 -- Q3/LConn1
  Q2/RConn1 -- DC minus/RConn1 -- Q4/RConn1
  Q2/LConn1 -- Q1/RConn1 -- Lf current/LConn1
  Q4/LConn1 -- Q3/RConn1 -- Cf/RConn1 -- Cf voltage/LConn2 -- Coil minus/RConn1
  Lf current/RConn1 -- Lf/LConn1
  Lf/RConn1 -- Lf resistance/LConn1
  Cp ESR/LConn1 -- Lf resistance/RConn1 -- Cf ESR/LConn1
  Cp/LConn1 -- Cp ESR/RConn1 -- Cp voltage/LConn1
  Coil plus/RConn1 -- Cp/RConn1 -- Cp voltage/LConn2
  Cf/LConn1 -- Cf ESR/RConn1 -- Cf voltage/LConn1

== system DWPT_DD_4section_100V/TX1 current ==
  Current Sensor : fl_lib/Electrical/Electrical Sensors/Current Sensor
  PS-Simulink Converter : nesl_utility/PS-Simulink Converter  PhysicalDomain=network_engine_domain  SubClassName=ps_output  LeftPortType=input  RightPortType=output  PseudoPeriodic=off  Frequencies=[]  VectorFormat=1-D array  Unit=A  AffineConversion=off
  + : PMIOPort  Side=Left
  - : PMIOPort  Port=2  Side=Right
  i : Outport  VectorParamsAs1DForOutWhenUnconnected=off
  wires:
  PS-Simulink Converter/1 -> i/1
  connections:
  PS-Simulink Converter/LConn1 -- Current Sensor/RConn1
  -/RConn1 -- Current Sensor/RConn2
  +/RConn1 -- Current Sensor/LConn1

== system DWPT_DD_4section_100V/TX2 current ==
  Current Sensor : fl_lib/Electrical/Electrical Sensors/Current Sensor
  PS-Simulink Converter : nesl_utility/PS-Simulink Converter  PhysicalDomain=network_engine_domain  SubClassName=ps_output  LeftPortType=input  RightPortType=output  PseudoPeriodic=off  Frequencies=[]  VectorFormat=1-D array  Unit=A  AffineConversion=off
  + : PMIOPort  Side=Left
  - : PMIOPort  Port=2  Side=Right
  i : Outport  VectorParamsAs1DForOutWhenUnconnected=off
  wires:
  PS-Simulink Converter/1 -> i/1
  connections:
  PS-Simulink Converter/LConn1 -- Current Sensor/RConn1
  -/RConn1 -- Current Sensor/RConn2
  +/RConn1 -- Current Sensor/LConn1

== system DWPT_DD_4section_100V/TX3 current ==
  Current Sensor : fl_lib/Electrical/Electrical Sensors/Current Sensor
  PS-Simulink Converter : nesl_utility/PS-Simulink Converter  PhysicalDomain=network_engine_domain  SubClassName=ps_output  LeftPortType=input  RightPortType=output  PseudoPeriodic=off  Frequencies=[]  VectorFormat=1-D array  Unit=A  AffineConversion=off
  + : PMIOPort  Side=Left
  - : PMIOPort  Port=2  Side=Right
  i : Outport  VectorParamsAs1DForOutWhenUnconnected=off
  wires:
  PS-Simulink Converter/1 -> i/1
  connections:
  PS-Simulink Converter/LConn1 -- Current Sensor/RConn1
  -/RConn1 -- Current Sensor/RConn2
  +/RConn1 -- Current Sensor/LConn1

== system DWPT_DD_4section_100V/TX4 current ==
  Current Sensor : fl_lib/Electrical/Electrical Sensors/Current Sensor
  PS-Simulink Converter : nesl_utility/PS-Simulink Converter  PhysicalDomain=network_engine_domain  SubClassName=ps_output  LeftPortType=input  RightPortType=output  PseudoPeriodic=off  Frequencies=[]  VectorFormat=1-D array  Unit=A  AffineConversion=off
  + : PMIOPort  Side=Left
  - : PMIOPort  Port=2  Side=Right
  i : Outport  VectorParamsAs1DForOutWhenUnconnected=off
  wires:
  PS-Simulink Converter/1 -> i/1
  connections:
  PS-Simulink Converter/LConn1 -- Current Sensor/RConn1
  -/RConn1 -- Current Sensor/RConn2
  +/RConn1 -- Current Sensor/LConn1

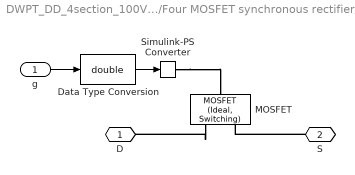
== system DWPT_DD_4section_100V/Four MOSFET synchronous rectifier/Q1 ==
  g : Inport
  Data Type Conversion : DataTypeConversion  OutDataTypeStr=double  SaturateOnIntegerOverflow=off  RndMeth=Floor
  MOSFET : ee_lib/Semiconductors & Converters/MOSFET (Ideal, Switching)  port_option=ee.enum.controlport.ps  Rds=RonSR Ohm  Goff=Goff 1/Ohm  Vth=0.5 V  diode_param=2  diode_Vf=bodyVf V  diode_Ron=bodyRon Ohm  diode_Goff=Goff 1/Ohm  diode_C=5e-8 F  diode_iRM=-235 A  diode_iF=300 A  diode_idot=-50 A/us  diode_trr_param=1  diode_trr_factor=3  diode_trr=15 us  diode_Qrr=1.5e+3 s*uA  ids_specify=off  ids_priority=None  ids=0 A  ids_nominal_specify=off  ids_nominal_value=1  ids_nominal_unit=A  vds_specify=off  vds_priority=None  vds=0 V  vds_nominal_specify=off  vds_nominal_value=1  vds_nominal_unit=V  vgs_specify=off  vgs_priority=None  vgs=0 V  vgs_nominal_specify=off  vgs_nominal_value=1  vgs_nominal_unit=V  thermal_loss_option=ee.enum.converters.thermalLossOption.constantvalues  Von_data=[0, 1.1, 1.3, 1.45, 1.75, 2.25, 2.7; 0, 1, 1.15, 1.35, 1.7, 2.35, 3] V  Tj=[298.15, 398.15] K  Iout_data=[0, 10, 50, 100, 200, 400, 600] A  tabulateWithVds=false  Eon_data=[0, .29, 1.43, 2.86, 5.71, 13.14, 22.86; 0, .57, 2.63, 5.14, 10.29, 20.57, 30.29] * 1e-3 J  Eoff_data=[0, .21, 1.07, 2.14, 4.29, 9.86, 17.14; 0, .43, 1.97, 3.86, 7.71, 15.43, 22.71] * 1e-3 J  Eon_data_3D=[zeros(2, 5, 3)] J  Eoff_data_3D=[zeros(2, 5, 3)] J  Tj_loss=[298.15, 448.15] K  Iout_data_loss=[0, 10, 20, 30, 40] A  Vds_loss=[0, 150, 300] V  Eon_scalar=22.86e-3 J  Eoff_scalar=17.14e-3 J  Voff=300 V  Iout_scalar=600 A  useCurrentFromPreviousCycle=true  currentMeasDelay=0 s  useVoltageFromPreviousCycle=true  voltageMeasDelay=0 s  diodeModelType=ee.enum.converters.diodeModelType.pwl  diodeTableType=ee.enum.diode.tableType.IfMat  diode_ReverseIVType=ee.enum.diode.diodeReverseIV.constant  diode_IfMat=[.07, .12, .19, 1.75, 4.24, 7.32, 11.2; .16, .3, .72, 2.14, 4.02, 6.35, 9.12] A  diode_VfMat=[.9, 1.15, 1.25, 1.5, 1.75, 2.17, 2.6, 2.85; .58, .68, .75, 1.1, 1.38, 1.77, 2.27, 2.7] V  diode_TjVec=[25, 125] degC  diode_VfVec=[.5, .7, .9, 1.3, 1.7, 2.1, 2.5] V  diode_IfVec=[.1, .2, .5, 1, 2, 4, 7, 10] A  diode_IrMat=[1e-06, 2e-06, 5e-06, 1e-05, 2.5e-05, 5e-05, .0001; 2e-06, 5e-06, 1e-05, 4e-05, 8e-05, .0002, .0005] A  diode_VrMat=[10, 100, 200, 250, 300, 325, 350; 10, 70, 160, 220, 270, 300, 320] V  diode_VrVec=[10, 20, 40, 50, 70, 80, 100] V  diode_IrVec=[1e-06, 2e-06, 5e-06, 1e-05, 2e-05, 5e-05, .0001] A  diode_Vr=-600 V  diode_Ls=150 nH  diode_Erec=0.03 J  diode_rec_loss_model=ee.enum.diode.reverseRecoveryModelTabulateUpTo3D.fixed  diode_ErecVal=0 J  diode_scaleWithIandV=true  diode_ErecMat=zeros(2, 3) J  diodeErecMat3D=zeros(2, 3, 2) J  diode_TjrecVec=[298.15, 398.15] K  diode_IfrecVec=[.1, 1, 10] A  diodeVrecVec=[0, 100] V  diode_IrecVal=10 A  diode_VrecVal=10 V  diode_tFilter=1 / 1000 / 100 s  separateThermalPortForDiode=false  thermal_network_parameterization=ee.enum.thermalNetworkTopology.external  Rth=[.03, .2] K/W  Rth_Cauer=[.03, .1, .2] K/W  Rth_Foster=[.03, .2] K/W  thermal_mass_parameterization=ee.enum.thermalNetwork.timeconstant  thermal_mass=[3, 25] J/K  thermal_mass_Cauer=[3, 10, 25] J/K  thermal_mass_Foster=[33, 50] J/K  thermal_time_constant=[.1, 5] s  thermal_time_constant_Cauer=[.1, 1, 5] s  thermal_time_constant_Foster=[1, 10] s  thermal_mass_initial_temperatures=[25, 25] degC  thermal_mass_initial_temperatures_Cauer=[25, 25, 25] degC  junction_thermal_mass=0.1 J/K  Tvec_initial_Foster=[25, 25, 25, 25] degC  RthDiode=[.03, .2] K/W  RthCauerDiode=[.03, .1, .2] K/W  RthFosterDiode=[.03, .2] K/W  thermalMassDiode=[3, 25] J/K  thermalMassCauerDiode=[3, 10, 25] J/K  thermalMassFosterDiode=[33, 50] J/K  thermalTauDiode=[.1, 5] s  thermalTauCauerDiode=[.1, 1, 5] s  thermalTauFosterDiode=[1, 10] s  thermalMassInitTempDiode=[25, 25] degC  thermalMassInitTempCauerDiode=[25, 25, 25] degC  junctionthermalMassDiode=0.1 J/K  TVecInitialFosterDiode=[25, 25] degC  no_thermal_network=ee.enum.enable.no  mosfet_junction_temperature_specify=off  mosfet_junction_temperature_priority=None  mosfet_junction_temperature=25 degC  mosfet_junction_temperature_nominal_specify=off  mosfet_junction_temperature_nominal_value=1  mosfet_junction_temperature_nominal_unit=degC  diode_junction_temperature_specify=off  diode_junction_temperature_priority=None  diode_junction_temperature=25 degC  diode_junction_temperature_nominal_specify=off  diode_junction_temperature_nominal_value=1  diode_junction_temperature_nominal_unit=degC  Qj_specify=off  Qj_priority=None  Qj=0 W  Qj_nominal_specify=off  Qj_nominal_value=1  Qj_nominal_unit=W  accumulatedSwitchingLosses_specify=off  accumulatedSwitchingLosses_priority=None  accumulatedSwitchingLosses=0 J
  Simulink-PS Converter : nesl_utility/Simulink-PS Converter  PhysicalDomain=network_engine_domain  SubClassName=ps_input  LeftPortType=input  RightPortType=output  PseudoPeriodic=off  Frequencies=[]  NoiseDistribution=none  NoiseParameters=[]  Unit=1  AffineConversion=off  FilteringAndDerivatives=provide  SimscapeFilterOrder=1  InputFilterTimeConstant=0.001  UdotUserProvided=0
  D : PMIOPort  Side=Left
  S : PMIOPort  Port=2  Side=Right
  wires:
  g/1 -> Data Type Conversion/1
  Data Type Conversion/1 -> Simulink-PS Converter/1
  connections:
  S/RConn1 -- MOSFET/RConn2
  Simulink-PS Converter/RConn1 -- MOSFET/LConn1
  MOSFET/RConn1 -- D/RConn1

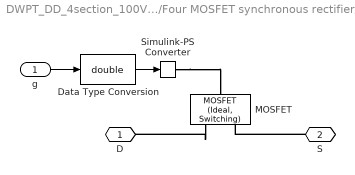
== system DWPT_DD_4section_100V/Four MOSFET synchronous rectifier/Q2 ==
  g : Inport
  Data Type Conversion : DataTypeConversion  OutDataTypeStr=double  SaturateOnIntegerOverflow=off  RndMeth=Floor
  MOSFET : ee_lib/Semiconductors & Converters/MOSFET (Ideal, Switching)  port_option=ee.enum.controlport.ps  Rds=RonSR Ohm  Goff=Goff 1/Ohm  Vth=0.5 V  diode_param=2  diode_Vf=bodyVf V  diode_Ron=bodyRon Ohm  diode_Goff=Goff 1/Ohm  diode_C=5e-8 F  diode_iRM=-235 A  diode_iF=300 A  diode_idot=-50 A/us  diode_trr_param=1  diode_trr_factor=3  diode_trr=15 us  diode_Qrr=1.5e+3 s*uA  ids_specify=off  ids_priority=None  ids=0 A  ids_nominal_specify=off  ids_nominal_value=1  ids_nominal_unit=A  vds_specify=off  vds_priority=None  vds=0 V  vds_nominal_specify=off  vds_nominal_value=1  vds_nominal_unit=V  vgs_specify=off  vgs_priority=None  vgs=0 V  vgs_nominal_specify=off  vgs_nominal_value=1  vgs_nominal_unit=V  thermal_loss_option=ee.enum.converters.thermalLossOption.constantvalues  Von_data=[0, 1.1, 1.3, 1.45, 1.75, 2.25, 2.7; 0, 1, 1.15, 1.35, 1.7, 2.35, 3] V  Tj=[298.15, 398.15] K  Iout_data=[0, 10, 50, 100, 200, 400, 600] A  tabulateWithVds=false  Eon_data=[0, .29, 1.43, 2.86, 5.71, 13.14, 22.86; 0, .57, 2.63, 5.14, 10.29, 20.57, 30.29] * 1e-3 J  Eoff_data=[0, .21, 1.07, 2.14, 4.29, 9.86, 17.14; 0, .43, 1.97, 3.86, 7.71, 15.43, 22.71] * 1e-3 J  Eon_data_3D=[zeros(2, 5, 3)] J  Eoff_data_3D=[zeros(2, 5, 3)] J  Tj_loss=[298.15, 448.15] K  Iout_data_loss=[0, 10, 20, 30, 40] A  Vds_loss=[0, 150, 300] V  Eon_scalar=22.86e-3 J  Eoff_scalar=17.14e-3 J  Voff=300 V  Iout_scalar=600 A  useCurrentFromPreviousCycle=true  currentMeasDelay=0 s  useVoltageFromPreviousCycle=true  voltageMeasDelay=0 s  diodeModelType=ee.enum.converters.diodeModelType.pwl  diodeTableType=ee.enum.diode.tableType.IfMat  diode_ReverseIVType=ee.enum.diode.diodeReverseIV.constant  diode_IfMat=[.07, .12, .19, 1.75, 4.24, 7.32, 11.2; .16, .3, .72, 2.14, 4.02, 6.35, 9.12] A  diode_VfMat=[.9, 1.15, 1.25, 1.5, 1.75, 2.17, 2.6, 2.85; .58, .68, .75, 1.1, 1.38, 1.77, 2.27, 2.7] V  diode_TjVec=[25, 125] degC  diode_VfVec=[.5, .7, .9, 1.3, 1.7, 2.1, 2.5] V  diode_IfVec=[.1, .2, .5, 1, 2, 4, 7, 10] A  diode_IrMat=[1e-06, 2e-06, 5e-06, 1e-05, 2.5e-05, 5e-05, .0001; 2e-06, 5e-06, 1e-05, 4e-05, 8e-05, .0002, .0005] A  diode_VrMat=[10, 100, 200, 250, 300, 325, 350; 10, 70, 160, 220, 270, 300, 320] V  diode_VrVec=[10, 20, 40, 50, 70, 80, 100] V  diode_IrVec=[1e-06, 2e-06, 5e-06, 1e-05, 2e-05, 5e-05, .0001] A  diode_Vr=-600 V  diode_Ls=150 nH  diode_Erec=0.03 J  diode_rec_loss_model=ee.enum.diode.reverseRecoveryModelTabulateUpTo3D.fixed  diode_ErecVal=0 J  diode_scaleWithIandV=true  diode_ErecMat=zeros(2, 3) J  diodeErecMat3D=zeros(2, 3, 2) J  diode_TjrecVec=[298.15, 398.15] K  diode_IfrecVec=[.1, 1, 10] A  diodeVrecVec=[0, 100] V  diode_IrecVal=10 A  diode_VrecVal=10 V  diode_tFilter=1 / 1000 / 100 s  separateThermalPortForDiode=false  thermal_network_parameterization=ee.enum.thermalNetworkTopology.external  Rth=[.03, .2] K/W  Rth_Cauer=[.03, .1, .2] K/W  Rth_Foster=[.03, .2] K/W  thermal_mass_parameterization=ee.enum.thermalNetwork.timeconstant  thermal_mass=[3, 25] J/K  thermal_mass_Cauer=[3, 10, 25] J/K  thermal_mass_Foster=[33, 50] J/K  thermal_time_constant=[.1, 5] s  thermal_time_constant_Cauer=[.1, 1, 5] s  thermal_time_constant_Foster=[1, 10] s  thermal_mass_initial_temperatures=[25, 25] degC  thermal_mass_initial_temperatures_Cauer=[25, 25, 25] degC  junction_thermal_mass=0.1 J/K  Tvec_initial_Foster=[25, 25, 25, 25] degC  RthDiode=[.03, .2] K/W  RthCauerDiode=[.03, .1, .2] K/W  RthFosterDiode=[.03, .2] K/W  thermalMassDiode=[3, 25] J/K  thermalMassCauerDiode=[3, 10, 25] J/K  thermalMassFosterDiode=[33, 50] J/K  thermalTauDiode=[.1, 5] s  thermalTauCauerDiode=[.1, 1, 5] s  thermalTauFosterDiode=[1, 10] s  thermalMassInitTempDiode=[25, 25] degC  thermalMassInitTempCauerDiode=[25, 25, 25] degC  junctionthermalMassDiode=0.1 J/K  TVecInitialFosterDiode=[25, 25] degC  no_thermal_network=ee.enum.enable.no  mosfet_junction_temperature_specify=off  mosfet_junction_temperature_priority=None  mosfet_junction_temperature=25 degC  mosfet_junction_temperature_nominal_specify=off  mosfet_junction_temperature_nominal_value=1  mosfet_junction_temperature_nominal_unit=degC  diode_junction_temperature_specify=off  diode_junction_temperature_priority=None  diode_junction_temperature=25 degC  diode_junction_temperature_nominal_specify=off  diode_junction_temperature_nominal_value=1  diode_junction_temperature_nominal_unit=degC  Qj_specify=off  Qj_priority=None  Qj=0 W  Qj_nominal_specify=off  Qj_nominal_value=1  Qj_nominal_unit=W  accumulatedSwitchingLosses_specify=off  accumulatedSwitchingLosses_priority=None  accumulatedSwitchingLosses=0 J
  Simulink-PS Converter : nesl_utility/Simulink-PS Converter  PhysicalDomain=network_engine_domain  SubClassName=ps_input  LeftPortType=input  RightPortType=output  PseudoPeriodic=off  Frequencies=[]  NoiseDistribution=none  NoiseParameters=[]  Unit=1  AffineConversion=off  FilteringAndDerivatives=provide  SimscapeFilterOrder=1  InputFilterTimeConstant=0.001  UdotUserProvided=0
  D : PMIOPort  Side=Left
  S : PMIOPort  Port=2  Side=Right
  wires:
  g/1 -> Data Type Conversion/1
  Data Type Conversion/1 -> Simulink-PS Converter/1
  connections:
  S/RConn1 -- MOSFET/RConn2
  Simulink-PS Converter/RConn1 -- MOSFET/LConn1
  MOSFET/RConn1 -- D/RConn1
